simulink model "controller"  (Simulink 7.0)
settings: Solver=FixedStepDiscrete  StartTime=0.0  StopTime=10.0  FixedStep=0.03  RelTol=1e-3
undefined symbols (not defined in the file or in its folder): OC1max
libraries: dsPICdrivers x7
settings Model: Creator=zhaosy  LastModifiedBy=zhaosy
settings OptimizationCC: OptimizeModelRefInitCode=on  LifeSpan=1
settings HardwareCC: ProdBitPerInt=16  ProdEndianess=LittleEndian  ProdWordSize=16  ProdHWDeviceType=16-bit Generic  TargetHWDeviceType=32-bit Generic
settings RTWCC: SystemTargetFile=dspic.tlc  TemplateMakefile=dspic_pic30_gcc.tmf  PostCodeGenCommand=dsPIC_Compile()  Description=Embedded Target for Microchip dsPIC (real-time)  ProcessScript=dspic_make_rtw_hook
settings CodeAppCC: IgnoreCustomStorageClasses=off
settings STFCustomTargetCC: GenFloatMathFcnCalls=ANSI_C  ModelReferenceCompliant=off  IncludeMdlTerminateFcn=off  CombineOutputUpdateFcns=on  SuppressErrorStatus=on  ERTCustomFileBanners=on  SupportContinuousTime=off  SupportNonInlinedSFcns=off  SystemTargetFile=dspic.tlc
settings ERTTargetCC: GenFloatMathFcnCalls=ANSI_C  ModelReferenceCompliant=off  CompOptLevelCompliant=off  IncludeMdlTerminateFcn=off  SuppressErrorStatus=on  ModelStepFunctionPrototypeControlCompliant=off  InlinedParameterPlacement=NonHierarchical  ERTSrcFileBannerTemplate=dsPIC_code_template.cgt  ERTHdrFileBannerTemplate=dsPIC_code_template.cgt  ERTDataSrcFileTemplate=dsPIC_code_template.cgt  ERTDataHdrFileTemplate=dsPIC_code_template.cgt  ERTCustomFileTemplate=dsPIC_main.tlc
settings CustomProperty: DataType=string  Value=C:\MATLAB\R2007b\bin\win32\gmake

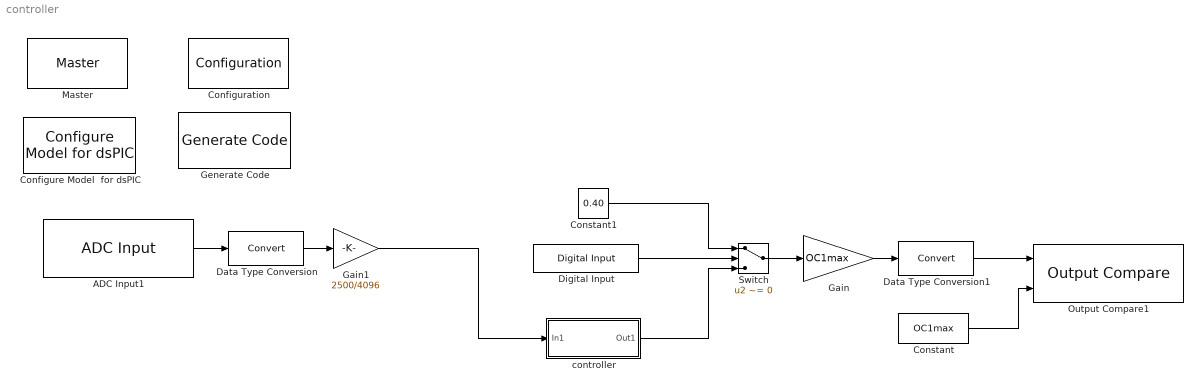
== system controller ==
  ADC Input1 : dsPICdrivers/Peripheral I//O/ADC Input  Tag=dsPIC_ADC  Priority=5  ADC_TYPE=12 bits  ADC_MODE=Continuous sampling & get last channel value  NbrSampleStep=1  VoltRefpopup="AVdd  -  AVss"  OutFormatBitspopup=0000 dddd dddd dddd : Integer  InterruptPriority=6  ANCHANNELS=[6]  MaxName=ANmax = 4096  Rin=0  ADCS=2  SAMC=1  Temperature=10  DMAChannel=0  SampleTime=-1  Status="OK  |  Tsmp=8.138e-007 |  T/Channel=1.221e-005 |  Tall=1.221e-005"
  Configuration : dsPICdrivers/Configuration  SystemSampleTime=-1  double64=on
  Configure Model  for dsPIC : dsPICdrivers/Simulink Configuration/Configure Model  for dsPIC
  Constant : Constant  Value=OC1max  OutDataTypeMode=uint16  OutDataType=sfix(16)  OutScaling=2^0  SampleTime=-1
  Constant1 : Constant  Value=0.40  OutDataTypeMode=double  OutDataType=fixdt(1,16,6)  ConRadixGroup=Best Precision: Vector-wise  SampleTime=-1
  Data Type Conversion : DataTypeConversion  OutDataTypeMode=double  OutDataType=sfix(16)  OutScaling=2^0
  Data Type Conversion1 : DataTypeConversion  OutDataTypeMode=uint16  OutDataType=sfix(16)  OutScaling=2^0
  Digital Input : dsPICdrivers/Digital I//O/Digital Input  Tag=dsPIC_Digital_Input  PORT=A  Pin=[12]  SampleTime=-1  OrderingInOutPopup=None
  Gain : Gain  Gain=OC1max  ParameterDataType=sfix(16)  ParameterScaling=2^0  OutDataTypeMode=double  OutDataType=sfix(16)  OutScaling=2^0
  Gain1 : Gain  Gain=2500/4096  ParameterDataType=sfix(16)  ParameterScaling=2^0  OutDataTypeMode=double  OutDataType=sfix(16)  OutScaling=2^0  SaturateOnIntegerOverflow=on
  Generate Code : dsPICdrivers/Simulink Configuration/Generate Code
  Master : dsPICdrivers/Master  Tag=dsPIC_MASTER  Priority=1  TimeStepType=Timer1  picType=30f6014  fcy=1843200  Quartz_33f=5e6  PLLActive_33f=off  fcyDesired_33f=0  tmr1="[1  55295  0]"  tmr1Info="Time Step : 0.03  ;   Error : 0%  PR1=55295"  tmr2345="[1  0  0  0]"  tmr2345cfg=[-1 -1 -1 -1]  IOautoConf=on  typePort="[ 0  0  0  0  0  0  0  0  0  0  0  0  9  0  0  0  0  0  0  0  0  0  8  0  0  0  0  0  0  0  0  0  0  0  0  0  0  0  0  0  0  0  0  0  0  0  0  0  7  0  0  0  0  0  0  0  0  0  0  0  0  0  0  0  0  0  0  0  0  0  0  0  0  0  0  0  0  0  0  0  0  0  0  0  0  0  0  0  0  0  0  0  0  0  0  0  0  0  0  0  0  0  0  0  0  0  0  0  0  0  0  0 ]"  TRIS="[ 65535  65535  65535  65534  65535  65535  65535 ]"  ADPCFG=0  MasterBusyPort=None  MasterOverloadPort=None  FOSC=HS  ClockSwitchMonitor=Both disabled  TempProtection_33f=TEMP_ON  FPBOR=PBOR_OFF  PWRT=PWRT_OFF  MCLR=MCLR_DIS  PowerSave=off  OverrideFcy=off  NewFcy=1e6
  Output Compare1 : dsPICdrivers/Peripheral I//O/Output Compare  Tag=dsPIC_PWM_out  Priority=5  IntPriority=3  CHANNEL=[1]  Channel_UP_Down_Periode=[5]  MaxChannel=[0.01333]  MaxName=' OC1max '  Precision=[14.5846]  Timer=[2]  Status=OK  SafeMarge=[0]  PortLetter=[68]  PortNumber=[0]  MaxValues=[24569.856]
  Switch : Switch  Criteria=u2 ~= 0  OutDataType=fixdt(1,16,6)
  controller : Subsystem  TreatAsAtomicUnit=on
  wires:
  Constant/1 -> Output Compare1/2
  Gain/1 -> Data Type Conversion1/1
  Constant1/1 -> Switch/1
  Digital Input/1 -> Switch/2
  controller/1(Out1) -> Switch/3
  Switch/1 -> Gain/1
  ADC Input1/1 -> Data Type Conversion/1
  Data Type Conversion/1 -> Gain1/1
  Gain1/1 -> controller/1(In1)
  Data Type Conversion1/1 -> Output Compare1/1

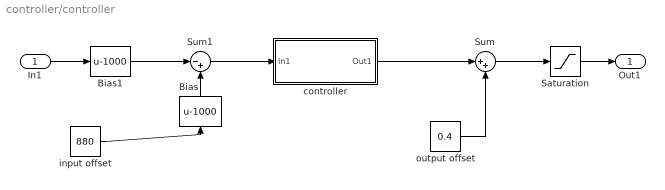
== system controller/controller ==
  In1 : Inport
  Bias : Bias  Orientation=up  Bias=-1000  SaturateOnIntegerOverflow=on
  Bias1 : Bias  Bias=-1000  SaturateOnIntegerOverflow=on
  Saturation : Saturate  UpperLimit=0.6  LowerLimit=0.1  OutDataTypeMode=double  OutDataType=fixdt(1,16,6)
  Sum : Sum  Inputs=|++  OutDataType=fixdt(1,16,6)
  Sum1 : Sum  Inputs=|-+  OutDataType=fixdt(1,16,3)
  controller : Subsystem
  input offset : Constant  Value=880  OutDataTypeMode=double  OutDataType=fixdt(1,16,3)  ConRadixGroup=Best Precision: Vector-wise  SampleTime=-1
  output offset : Constant  Value=0.4  OutDataTypeMode=double  OutDataType=fixdt(1,16,6)  ConRadixGroup=Best Precision: Vector-wise  SampleTime=-1
  Out1 : Outport  OutDataType=sfix(16)  OutScaling=2^0
  wires:
  Sum/1 -> Saturation/1
  output offset/1 -> Sum/2
  input offset/1 -> Bias/1
  In1/1 -> Bias1/1
  Bias1/1 -> Sum1/1
  Bias/1 -> Sum1/2
  controller/1(Out1) -> Sum/1
  Sum1/1 -> controller/1(In1)
  Saturation/1 -> Out1/1

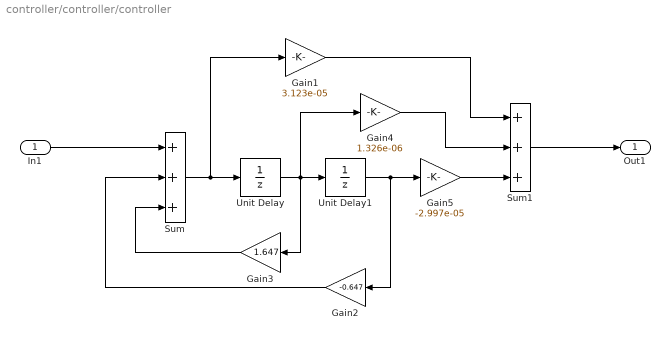
== system controller/controller/controller ==
  In1 : Inport  OutDataType=sfix(16)  OutScaling=2^0
  Gain1 : Gain  Gain=3.123e-05  ParameterDataType=sfix(32)  OutDataTypeMode=double  OutDataType=fixdt(1,64,32)  SaturateOnIntegerOverflow=on
  Gain2 : Gain  Orientation=left  Gain=-0.647  ParameterDataType=sfix(32)  OutDataTypeMode=double  OutDataType=fixdt(1,32,16)  SaturateOnIntegerOverflow=on
  Gain3 : Gain  Orientation=left  Gain=1.647  ParameterDataType=sfix(32)  OutDataTypeMode=double  OutDataType=fixdt(1,32,16)  SaturateOnIntegerOverflow=on
  Gain4 : Gain  Gain=1.326e-06  ParameterDataType=sfix(32)  OutDataTypeMode=double  OutDataType=fixdt(1,32,16)  SaturateOnIntegerOverflow=on
  Gain5 : Gain  Gain=-2.997e-05  ParameterDataType=sfix(32)  OutDataTypeMode=double  OutDataType=fixdt(1,32,16)  SaturateOnIntegerOverflow=on
  Sum : Sum  Inputs=+++  OutDataTypeMode=double  OutDataType=fixdt(1,64,32)  SampleTime=0.03
  Sum1 : Sum  Inputs=+++  OutDataTypeMode=double  OutDataType=fixdt(1,64,32)  SampleTime=0.03
  Unit Delay : UnitDelay  X0=0.0  SampleTime=-1
  Unit Delay1 : UnitDelay  X0=0.0  SampleTime=-1
  Out1 : Outport  OutDataType=sfix(16)  OutScaling=2^0
  wires:
  Gain3/1 -> Sum/3
  Gain1/1 -> Sum1/1
  Sum1/1 -> Out1/1
  In1/1 -> Sum/1
  Sum/1 -> Unit Delay/1, Gain1/1
  Gain5/1 -> Sum1/3
  Gain4/1 -> Sum1/2
  Unit Delay/1 -> Gain3/1, Unit Delay1/1, Gain4/1
  Gain2/1 -> Sum/2
  Unit Delay1/1 -> Gain5/1, Gain2/1
